simulink model "W07_pose_dp"  (R2024b)
settings: Solver=ode4  StartTime=0  StopTime=T_pose  FixedStep=h  RelTol=1e-3
InitFcn:
  | addpath(fullfile(fileparts(fileparts(fileparts(get_param(bdroot, 'FileName')))), '_tools'), fileparts(get_param(bdroot, 'FileName'))); run_alone('W07', bdroot);
StopFcn:
  | W07_plot_pose;
values from neighbouring files (symbols this model uses):
  alpha_lim = cfg.alpha_max(1)    [W07_0_setup.m]
  animate = 1    [W07_0_setup.m]    (also in W07_alloc_run.m = 0; W07_pose_run.m = 0; W07_wpt_run.m = 0)
  B_alloc = cfg.B    [W07_0_setup.m]
  beta_c = pi/2    (= 1.57079632679)    [W07_0_setup.m]
  eps_reg = 1e-4    (= 0.0001)    [W07_0_setup.m]    (also in W07_alloc_run.m)
  h = 0.02    [W07_0_setup.m]    (also in W07_3_build_wpt.m = add_line(sys, [a; via; b]); W07_4_build_pose.m = add_line(sys, [a; via; b]))
  k_neg = cfg.k_neg    [W07_0_setup.m]
  k_pos = cfg.k_pos    [W07_0_setup.m]
  Kb = 1    [W07_0_setup.m]
  Kd = 100    [W07_0_setup.m]
  Ki_u = 200    [W07_0_setup.m]
  Ki_v = 200    [W07_0_setup.m]
  Kp = 300    [W07_0_setup.m]
  Kp_pos = 0.30    (= 0.3)    [W07_0_setup.m]
  Kp_u = 200    [W07_0_setup.m]
  Kp_v = 200    [W07_0_setup.m]
  mp = 25    [W07_0_setup.m]
  N_lim = 150    [W07_0_setup.m]
  n_max = cfg.n_max    [W07_0_setup.m]    (also in W07_plot_ca.m = base_num('n_max',      103.93); W07_plot_sat.m = base_var('n_max',      103.931))
  n_min = cfg.n_min    [W07_0_setup.m]    (also in W07_plot_ca.m = base_num('n_min',     -101.74); W07_plot_sat.m = base_var('n_min',     -101.737))
  p_d = [10; 10]    [W07_0_setup.m]
  psi_set = deg2rad(45)    [W07_0_setup.m]
  Q_tau = eye(3)    [W07_0_setup.m]    (also in W07_alloc_run.m)
  quad = [cfg.pos ; cfg.alpha_max ; cfg.mount]    [W07_0_setup.m]
  rp = [0.05 0 -0.35]'    [W07_0_setup.m]
  T_neg = cfg.k_neg * cfg.n_min^2    [W07_0_setup.m]    (also in W07_plot_ca.m = base_num('T_neg',       66.708); W07_plot_sat.m = base_var('T_neg',        66.708))
  T_pos = cfg.k_pos * cfg.n_max^2    [W07_0_setup.m]    (also in W07_plot_ca.m = base_num('T_pos',      119.682); W07_plot_sat.m = base_var('T_pos',       119.682))
  u_lim = 0.80    (= 0.8)    [W07_0_setup.m]
  V_c = 0.0    (= 0)    [W07_0_setup.m]
  v_lim = 0.60    (= 0.6)    [W07_0_setup.m]
  W_alloc = diag(repmat([1 10], 1, 4))    [W07_0_setup.m]
  x0 = zeros(12,1)    [W07_0_setup.m]
  X_max = 120    [W07_0_setup.m]
  Y_max = 120    [W07_0_setup.m]
settings Model: Creator=admin  LastModifiedBy=admin
settings DataIOCC: ReturnWorkspaceOutputs=off

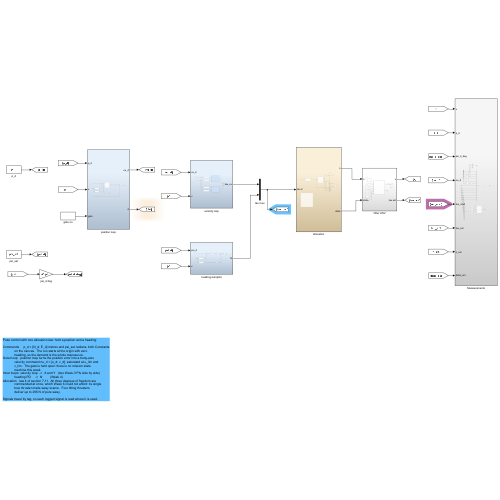
[thumbnail: Simulink's stored preview of the top-level diagram]
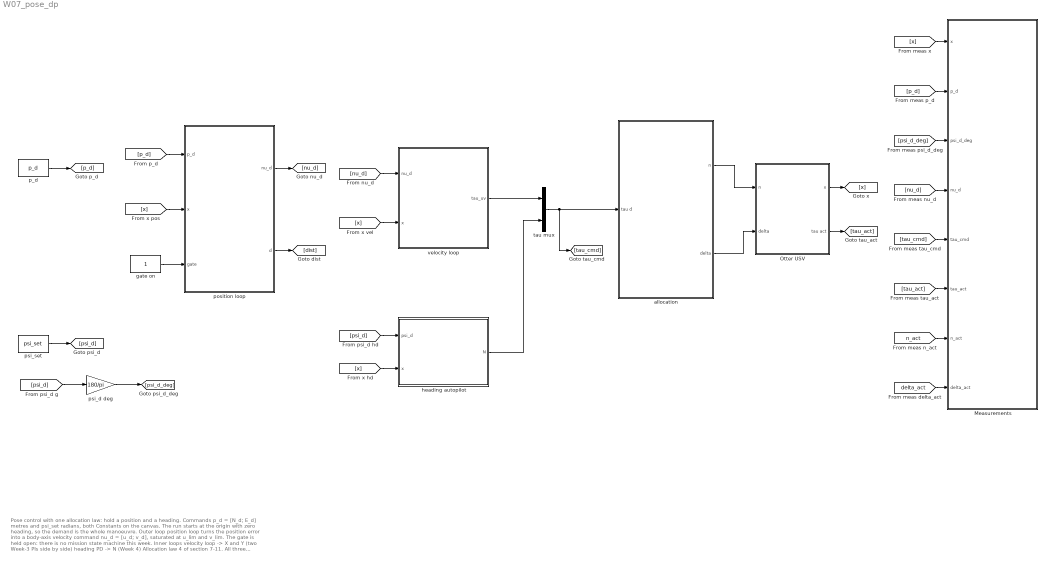
== system W07_pose_dp ==
  note: Pose control with one allocation law: hold a position and a heading.
      |
      | Commands     p_d = [N_d; E_d] metres and psi_set radians, both Constants
      |              on the canvas.  The run starts at the origin with zero
      |              heading, so the demand is the whole manoeuvre.
      | Outer loop   position loop turns the position error into a body-axis
      |              velocity command nu_d = [u_d; v_d], saturated at u_lim and
      |              v_lim.  The gate is held open: there is no mission state
      |              machine this week.
      | Inner loops  velocity loop  ->  X and Y   (two Week-3 PIs side by side)
      |              heading PD     ->  N         (Week 4)
      | Allocation   law 4 of section 7-11.  All three degrees of freedom are
      |              commanded at once, which Week 6 could not afford: its single
      |              bow thruster made sway scarce.  Four tilting thrusters
      |              deliver up to 295 N of pure sway.
      |
      | Signals travel by tag, so each logged signal is read where it is used.
  Measurements : Subsystem
  Otter USV : Subsystem
  allocation : Subsystem
  gate on : Constant
  heading autopilot : Subsystem
  p_d : Constant  Value=p_d
  position loop : Subsystem
  psi_d deg : Gain  Gain=180/pi
  psi_set : Constant  Value=psi_set
  tau mux : Mux  Inputs=2
  velocity loop : Subsystem
  wires:
  p_d/1 -> [p_d]
  psi_set/1 -> [psi_d]
  [psi_d] -> psi_d deg/1
  psi_d deg/1 -> [psi_d_deg]
  [p_d] -> position loop/1(p_d)
  [x] -> position loop/2(x)
  gate on/1 -> position loop/3(gate)
  position loop/1(nu_d) -> [nu_d]
  position loop/2(d) -> [dist]
  [nu_d] -> velocity loop/1(nu_d)
  [x] -> velocity loop/2(x)
  [psi_d] -> heading autopilot/1(psi_d)
  [x] -> heading autopilot/2(x)
  velocity loop/1(tau_uv) -> tau mux/1
  heading autopilot/1(N) -> tau mux/2
  tau mux/1 -> [tau_cmd], allocation/1(tau d)
  allocation/1(n) -> Otter USV/1(n)
  allocation/2(delta) -> Otter USV/2(delta)
  Otter USV/1(x) -> [x]
  Otter USV/2(tau act) -> [tau_act]
  [x] -> Measurements/1(x)
  [p_d] -> Measurements/2(p_d)
  [psi_d_deg] -> Measurements/3(psi_d_deg)
  [nu_d] -> Measurements/4(nu_d)
  [tau_cmd] -> Measurements/5(tau_cmd)
  [tau_act] -> Measurements/6(tau_act)
  [n_act] -> Measurements/7(n_act)
  [delta_act] -> Measurements/8(delta_act)

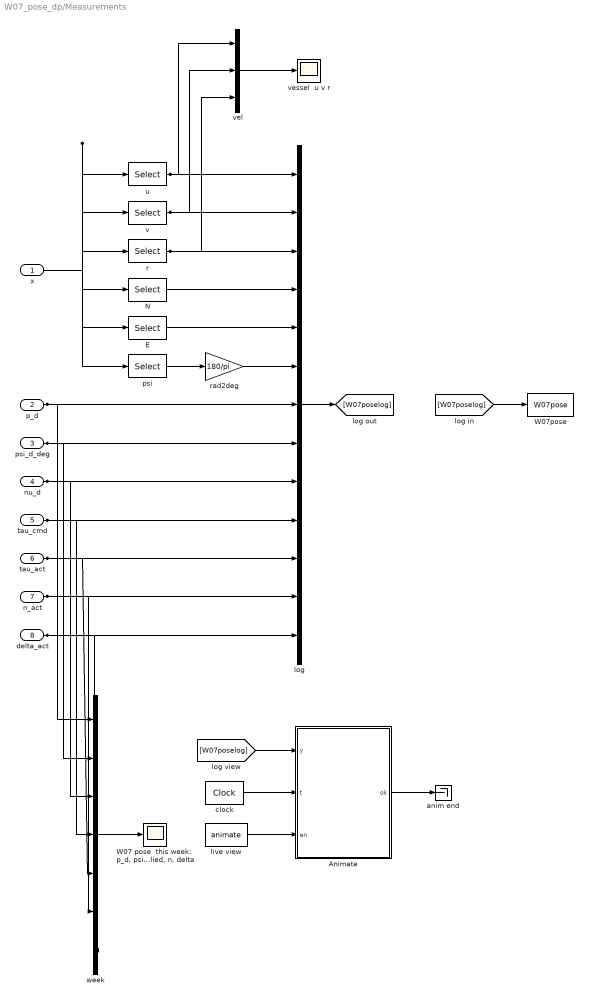
== system W07_pose_dp/Measurements ==
  x : Inport
  p_d : Inport  Port=2
  psi_d_deg : Inport  Port=3
  nu_d : Inport  Port=4
  tau_cmd : Inport  Port=5
  tau_act : Inport  Port=6
  n_act : Inport  Port=7
  delta_act : Inport  Port=8
  Animate : MATLAB Function  TreatAsAtomicUnit=on
  E : Selector  InputPortWidth=12  IndexOptions=Index vector (dialog)  Indices=8  OutputSizes=1
  N : Selector  InputPortWidth=12  IndexOptions=Index vector (dialog)  Indices=7  OutputSizes=1
  "W07 pose  this week:  p_d, psi_d, nu_d, tau asked and applied, n, delta" : Scope
  W07pose : ToWorkspace  VariableName=W07pose  SaveFormat=Structure With Time  SampleTime=-1
  anim end : Terminator
  clock : DigitalClock  SampleTime=h
  live view : Constant  Value=animate
  log : Mux  Inputs=13
  psi : Selector  InputPortWidth=12  IndexOptions=Index vector (dialog)  Indices=12  OutputSizes=1
  r : Selector  InputPortWidth=12  IndexOptions=Index vector (dialog)  Indices=6  OutputSizes=1
  rad2deg : Gain  Gain=180/pi
  u : Selector  InputPortWidth=12  IndexOptions=Index vector (dialog)  Indices=1  OutputSizes=1
  v : Selector  InputPortWidth=12  IndexOptions=Index vector (dialog)  Indices=2  OutputSizes=1
  vel : Mux  Inputs=3
  vessel  u v r : Scope
  week : Mux  Inputs=7
  wires:
  x/1 -> u/1, v/1, r/1, N/1, E/1, psi/1
  log/1 -> [W07poselog]
  [W07poselog] -> W07pose/1
  psi/1 -> rad2deg/1
  u/1 -> log/1, vel/1
  v/1 -> log/2, vel/2
  r/1 -> log/3, vel/3
  N/1 -> log/4
  E/1 -> log/5
  rad2deg/1 -> log/6
  p_d/1 -> log/7, week/1
  psi_d_deg/1 -> log/8, week/2
  nu_d/1 -> log/9, week/3
  tau_cmd/1 -> log/10, week/4
  tau_act/1 -> log/11, week/5
  n_act/1 -> log/12, week/6
  delta_act/1 -> log/13, week/7
  vel/1 -> vessel  u v r/1
  week/1 -> "W07 pose  this week:  p_d, psi_d, nu_d, tau asked and applied, n, delta"/1
  [W07poselog] -> Animate/1(y)
  clock/1 -> Animate/2(t)
  live view/1 -> Animate/3(en)
  Animate/1(ok) -> anim end/1

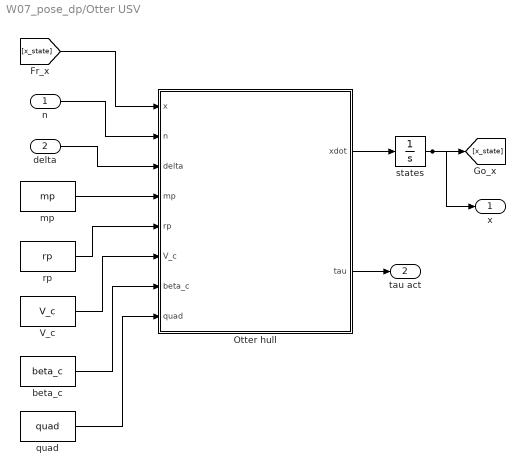
== system W07_pose_dp/Otter USV ==
  n : Inport
  delta : Inport  Port=2
  Otter hull : MATLAB Function  TreatAsAtomicUnit=on
  V_c : Constant  Value=V_c
  beta_c : Constant  Value=beta_c
  mp : Constant  Value=mp
  quad : Constant  Value=quad
  rp : Constant  Value=rp
  states : Integrator  InitialCondition=x0
  x : Outport
  tau act : Outport  Port=2
  wires:
  n/1 -> Otter hull/2(n)
  [x_state] -> Otter hull/1(x)
  delta/1 -> Otter hull/3(delta)
  mp/1 -> Otter hull/4(mp)
  rp/1 -> Otter hull/5(rp)
  V_c/1 -> Otter hull/6(V_c)
  beta_c/1 -> Otter hull/7(beta_c)
  quad/1 -> Otter hull/8(quad)
  Otter hull/1(xdot) -> states/1
  Otter hull/2(tau) -> tau act/1
  states/1 -> [x_state], x/1

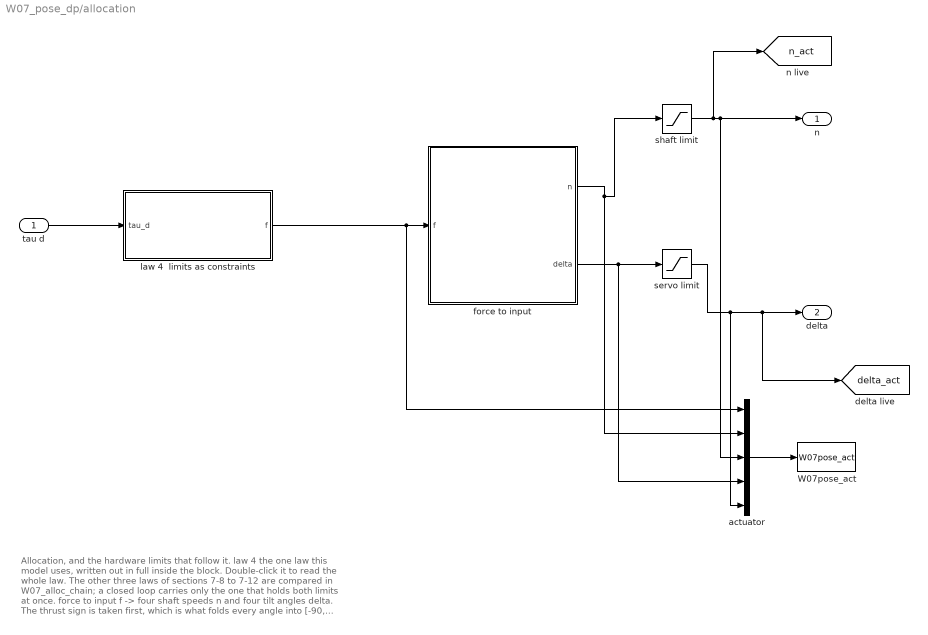
== system W07_pose_dp/allocation ==
  note: Allocation, and the hardware limits that follow it.
      |
      | law 4             the one law this model uses, written out in full
      |                   inside the block. Double-click it to read the whole law.
      |                   The other three laws of sections 7-8 to 7-12 are compared
      |                   in W07_alloc_chain; a closed loop carries only the one
      |                   that holds both limits at once.
      | force to input    f -> four shaft speeds n and four tilt angles delta. The
      |                   thrust sign is taken first, which is what folds every
      |                   angle into [-90, +90] deg before the servo ever sees it.
      |                   A unit asked for less than 0.5 N is held at n = 0 and
      |                   delta = 0, because below that the angle is arithmetic
      |                   noise and the servo would chatter at rest.
      | shaft limit       n clipped to [n_min, n_max].
      | servo limit       delta clipped to +-alpha_lim.
      | n live            the two clipped commands also leave as the global tags
      | delta live        n_act and delta_act, so the live view can draw them
      |                   against their limits while the run is still going. The
      |                   record below is readable only after it ends.
      | actuator          the record of this solve, written to W07pose_act as 24
      |                   columns:  f(8),  n asked(4),  n allowed(4),  delta
      |                   asked(4),  delta allowed(4). Wherever asked and allowed
      |                   differ, that unit is against a limit.
      |
      | What the hull was actually given is not rebuilt here: the motion model
      | already forms it from the clipped n and delta and reports it on its own
      | second output.
  tau d : Inport
  W07pose_act : ToWorkspace  VariableName=W07pose_act  SampleTime=-1
  actuator : Mux  Inputs=5
  force to input : MATLAB Function  TreatAsAtomicUnit=on
  law 4  limits as constraints : MATLAB Function  TreatAsAtomicUnit=on
  servo limit : Saturate  UpperLimit=alpha_lim  LowerLimit=-alpha_lim
  shaft limit : Saturate  UpperLimit=n_max  LowerLimit=n_min
  n : Outport
  delta : Outport  Port=2
  tag scope: delta_act=global, n_act=global
  wires:
  tau d/1 -> law 4  limits as constraints/1(tau_d)
  law 4  limits as constraints/1(f) -> force to input/1(f), actuator/1
  force to input/1(n) -> shaft limit/1, actuator/2
  force to input/2(delta) -> actuator/4, servo limit/1
  shaft limit/1 -> n/1, actuator/3, [n_act]
  servo limit/1 -> [delta_act], delta/1, actuator/5
  actuator/1 -> W07pose_act/1

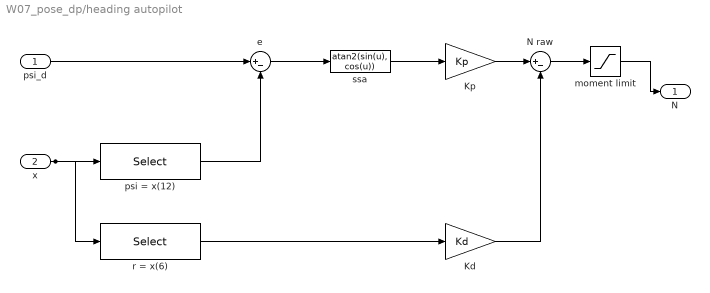
== system W07_pose_dp/heading autopilot ==
  psi_d : Inport
  x : Inport  Port=2
  Kd : Gain  Gain=Kd
  Kp : Gain  Gain=Kp
  N raw : Sum  Inputs=|+-
  e : Sum  Inputs=|+-
  moment limit : Saturate  UpperLimit=N_lim  LowerLimit=-N_lim
  psi = x(12) : Selector  InputPortWidth=12  IndexOptions=Index vector (dialog)  Indices=12  OutputSizes=1
  r = x(6) : Selector  InputPortWidth=12  IndexOptions=Index vector (dialog)  Indices=6  OutputSizes=1
  ssa : Fcn  Expr=atan2(sin(u), cos(u))
  N : Outport
  wires:
  x/1 -> psi = x(12)/1, r = x(6)/1
  psi_d/1 -> e/1
  psi = x(12)/1 -> e/2
  e/1 -> ssa/1
  ssa/1 -> Kp/1
  r = x(6)/1 -> Kd/1
  Kp/1 -> N raw/1
  Kd/1 -> N raw/2
  N raw/1 -> moment limit/1
  moment limit/1 -> N/1

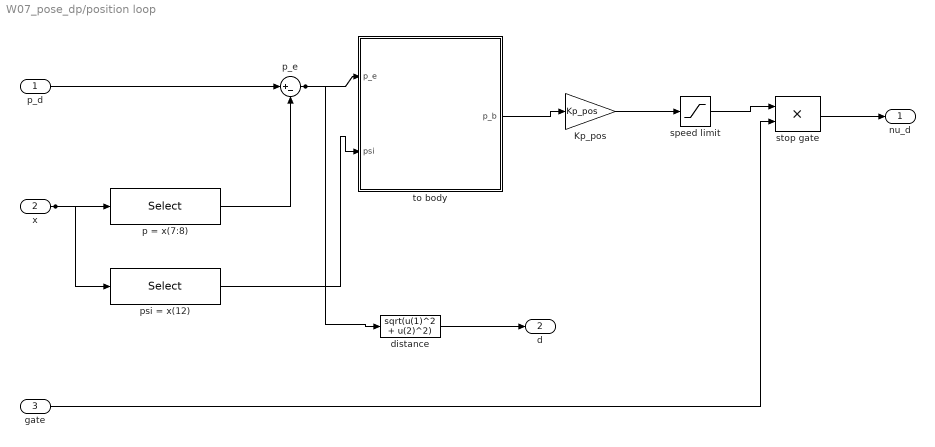
== system W07_pose_dp/position loop ==
  p_d : Inport
  x : Inport  Port=2
  gate : Inport  Port=3
  Kp_pos : Gain  Gain=Kp_pos
  distance : Fcn  Expr=sqrt(u(1)^2 + u(2)^2)
  p = x(7:8) : Selector  InputPortWidth=12  IndexOptions=Index vector (dialog)  Indices=[7 8]  OutputSizes=1
  p_e : Sum  Inputs=|+-
  psi = x(12) : Selector  InputPortWidth=12  IndexOptions=Index vector (dialog)  Indices=12  OutputSizes=1
  speed limit : Saturate  UpperLimit="[ u_lim;  v_lim]"  LowerLimit=[-u_lim; -v_lim]
  stop gate : Product
  to body : MATLAB Function  TreatAsAtomicUnit=on
  nu_d : Outport
  d : Outport  Port=2
  wires:
  x/1 -> p = x(7:8)/1, psi = x(12)/1
  p_d/1 -> p_e/1
  p = x(7:8)/1 -> p_e/2
  p_e/1 -> to body/1(p_e), distance/1
  psi = x(12)/1 -> to body/2(psi)
  to body/1(p_b) -> Kp_pos/1
  Kp_pos/1 -> speed limit/1
  speed limit/1 -> stop gate/1
  gate/1 -> stop gate/2
  stop gate/1 -> nu_d/1
  distance/1 -> d/1

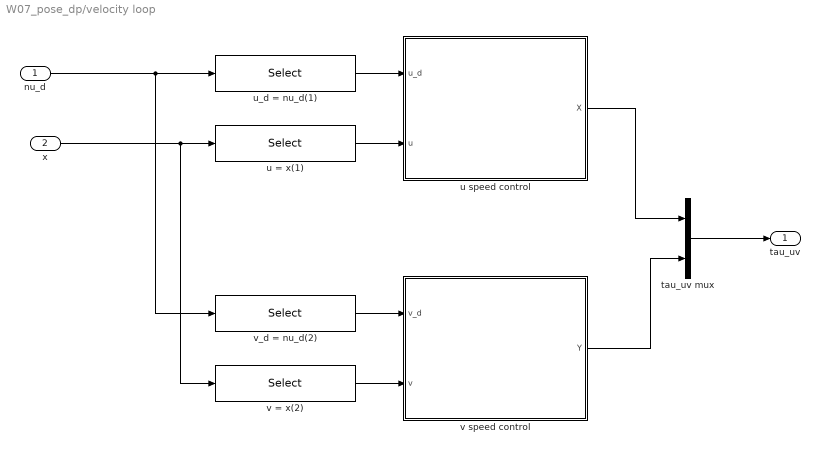
== system W07_pose_dp/velocity loop ==
  nu_d : Inport
  x : Inport  Port=2
  tau_uv mux : Mux  Inputs=2
  u = x(1) : Selector  InputPortWidth=12  IndexOptions=Index vector (dialog)  Indices=1  OutputSizes=1
  u speed control : Subsystem
  u_d = nu_d(1) : Selector  InputPortWidth=2  IndexOptions=Index vector (dialog)  Indices=1  OutputSizes=1
  v = x(2) : Selector  InputPortWidth=12  IndexOptions=Index vector (dialog)  Indices=2  OutputSizes=1
  v speed control : Subsystem
  v_d = nu_d(2) : Selector  InputPortWidth=2  IndexOptions=Index vector (dialog)  Indices=2  OutputSizes=1
  tau_uv : Outport
  wires:
  u_d = nu_d(1)/1 -> u speed control/1(u_d)
  u = x(1)/1 -> u speed control/2(u)
  v_d = nu_d(2)/1 -> v speed control/1(v_d)
  v = x(2)/1 -> v speed control/2(v)
  nu_d/1 -> u_d = nu_d(1)/1, v_d = nu_d(2)/1
  x/1 -> u = x(1)/1, v = x(2)/1
  u speed control/1(X) -> tau_uv mux/1
  v speed control/1(Y) -> tau_uv mux/2
  tau_uv mux/1 -> tau_uv/1

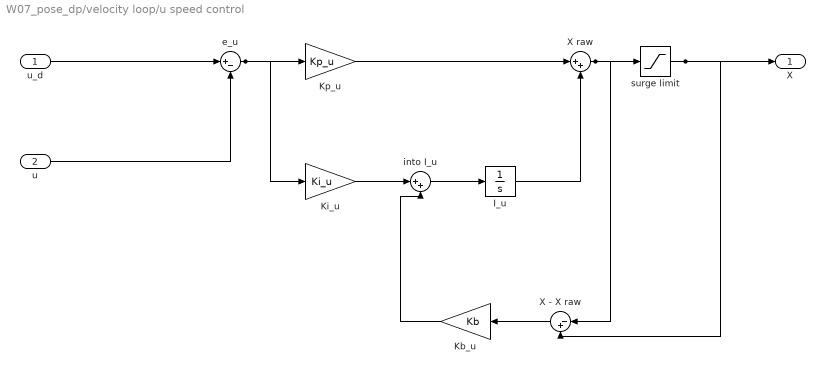
== system W07_pose_dp/velocity loop/u speed control ==
  u_d : Inport
  u : Inport  Port=2
  I_u : Integrator
  Kb_u : Gain  Gain=Kb
  Ki_u : Gain  Gain=Ki_u
  Kp_u : Gain  Gain=Kp_u
  X - X raw : Sum  Inputs=|-+
  X raw : Sum  Inputs=|++
  e_u : Sum  Inputs=|+-
  into I_u : Sum  Inputs=|++
  surge limit : Saturate  UpperLimit=X_max  LowerLimit=-X_max
  X : Outport
  wires:
  u_d/1 -> e_u/1
  u/1 -> e_u/2
  e_u/1 -> Kp_u/1, Ki_u/1
  Ki_u/1 -> into I_u/1
  into I_u/1 -> I_u/1
  Kp_u/1 -> X raw/1
  I_u/1 -> X raw/2
  X raw/1 -> surge limit/1, X - X raw/1
  surge limit/1 -> X - X raw/2, X/1
  X - X raw/1 -> Kb_u/1
  Kb_u/1 -> into I_u/2

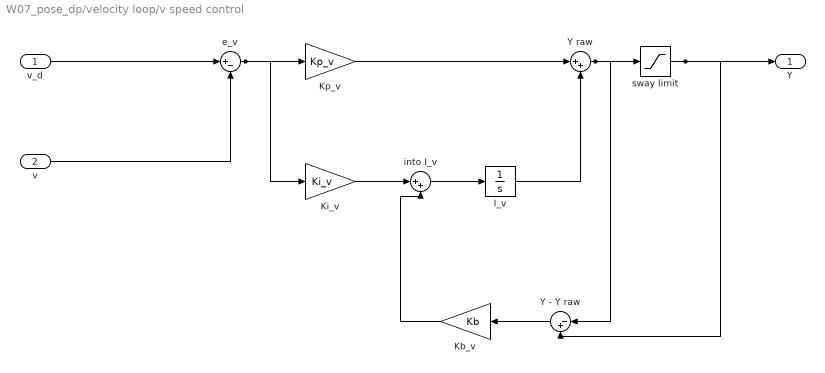
== system W07_pose_dp/velocity loop/v speed control ==
  v_d : Inport
  v : Inport  Port=2
  I_v : Integrator
  Kb_v : Gain  Gain=Kb
  Ki_v : Gain  Gain=Ki_v
  Kp_v : Gain  Gain=Kp_v
  Y - Y raw : Sum  Inputs=|-+
  Y raw : Sum  Inputs=|++
  e_v : Sum  Inputs=|+-
  into I_v : Sum  Inputs=|++
  sway limit : Saturate  UpperLimit=Y_max  LowerLimit=-Y_max
  Y : Outport
  wires:
  v_d/1 -> e_v/1
  v/1 -> e_v/2
  e_v/1 -> Kp_v/1, Ki_v/1
  Ki_v/1 -> into I_v/1
  into I_v/1 -> I_v/1
  Kp_v/1 -> Y raw/1
  I_v/1 -> Y raw/2
  Y raw/1 -> sway limit/1, Y - Y raw/1
  sway limit/1 -> Y - Y raw/2, Y/1
  Y - Y raw/1 -> Kb_v/1
  Kb_v/1 -> into I_v/2

== matlab function W07_pose_dp/allocation/law 4  limits as constraints ==
  data: tau_d input; f output double size=[8 1]; B_alloc parameter; W_alloc parameter; alpha_lim parameter; Q_tau parameter; eps_reg parameter; T_pos parameter; T_neg parameter
function f = law4_limits_as_constraints(tau_d, B_alloc, W_alloc, alpha_lim, Q_tau, eps_reg, T_pos, T_neg)
% LAW 4 -- the servo limit AND the thrust cap as hard constraints.  7-12.
%
% Minimise   ||Q (B f - tau_d)||^2 + eps ||W^(1/2) f||^2
% subject to, for every unit i,
%
%     |f_yi| <= tan(alpha_lim) sigma_i f_xi               the servo limit
%     cos(th) x' + sin(th) y' <= R cos(alpha_lim/M)       the thrust cap
%
% written in unit axes x' = sigma_i f_xi and y' = sigma_i f_yi. Both are
% straight lines once the thrust sign sigma_i of that unit is fixed, so the
% problem is a QP: no local minima. The signs are not known in advance, so
% all 2^4 = 16 sign combinations are solved and the cheapest feasible one is
% kept. tau_d sits in the cost rather than in an equality, so a solution
% exists even when the demand cannot be delivered.
%
% The cap is an arc, which no QP can hold. It is replaced by M = 3 inscribed
% chords: neighbouring chords meet exactly on the circle of radius R and
% their midpoints sit at cos(15 deg) = 0.966 R, so the polygon never breaks
% the cap and is at worst 3.4 per cent conservative.
%
% lsqlin has no code generation support, so the call is extrinsic and every
% output it returns is given a size and a type beforehand.
coder.extrinsic('lsqlin', 'optimoptions');

M = 3;                   % chords per cone, the n_chord of W07_vars
t = tan(alpha_lim);

% the whole cost as one least-squares residual,  ||C f - d||
C = [Q_tau*B_alloc ; sqrt(eps_reg)*sqrt(W_alloc)];
d = [Q_tau*tau_d   ; zeros(8,1)];

% the fallback, used if no sign combination turns out to be feasible
Wi = W_alloc \ eye(8);
f  = Wi * B_alloc' * ((B_alloc*Wi*B_alloc') \ tau_d);

opts = optimoptions('lsqlin', 'Display', 'off');
best = inf;

for p = 0:15
    % the four thrust signs of combination p, read off its four bits
    sg = zeros(4,1);
    for i = 1:4
        sg(i) = 1 - 2*mod(floor(p/2^(i-1)), 2);
    end

    A = zeros(4*(2+M), 8);
    b = zeros(4*(2+M), 1);
    r = 0;
    for i = 1:4
        s = sg(i);
        if s > 0
            R = T_pos;
        else
            R = T_neg;    % written positive, so the cap is a radius
        end
        r = r + 1;  A(r, 2*i-1) = -t*s;  A(r, 2*i) =  1;
        r = r + 1;  A(r, 2*i-1) = -t*s;  A(r, 2*i) = -1;
        for j = 1:M
            th = -alpha_lim + (j - 0.5)*(2*alpha_lim/M);
            r  = r + 1;
            A(r, 2*i-1) = s*cos(th);
            A(r, 2*i)   = s*sin(th);
            b(r)        = R*cos(alpha_lim/M);
        end
    end

    x   = zeros(8,1);
    cst = 0;
    res = zeros(11,1);
    ef  = 0;
    [x, cst, res, ef] = lsqlin(C, d, A, b, [], [], [], [], [], opts);

    % a cost is a cost only where the solver reported a solution
    if ef > 0 && cst < best
        best = cst;
        f    = x;
    end
end
end

== matlab function W07_pose_dp/position loop/to body ==
  data: p_e input; p_b output double size=[2 1]; psi input
function p_b = to_body(p_e, psi)
% Rotate the position error from NED into the body frame.
%
%            [ cos(psi)  -sin(psi) ]
%   R(psi) = [ sin(psi)   cos(psi) ]     maps the BODY frame to NED,
%
% so the transpose maps NED to the body frame. R is orthogonal, so the
% transpose is the inverse and nothing is lost in the change of frame: the
% distance to the target is the same number in either one.
c = cos(psi);
s = sin(psi);
p_b = [  c*p_e(1) + s*p_e(2) ;      % 전진 방향의 오차 / along the bow
        -s*p_e(1) + c*p_e(2) ];     % 우현 방향의 오차 / to starboard
end

== matlab function W07_pose_dp/allocation/force to input ==
  data: f input; n output double size=[4 1]; delta output; k_pos parameter; k_neg parameter
function [n, delta] = force2input(f, k_pos, k_neg)
% Eight force components -> four shaft speeds and four tilt angles.
%
%     sigma_i = sign(f_xi)                        which way the unit pushes
%     T_i     = sigma_i |f_i|                     signed thrust        [N]
%     delta_i = atan2(sigma_i f_yi, sigma_i f_xi) tilt angle         [rad]
%     n_i     = sign(T_i) sqrt(|T_i| / k_i)       shaft speed      [rad/s]
%
% Multiplying BOTH arguments of atan2 by sigma_i turns the direction through
% exactly pi, and because sigma_i f_xi >= 0 the result always lands in
% [-pi/2, +pi/2]. That is what keeps the angle reachable: a unit pushing
% astern comes out as negative thrust at a small angle instead of positive
% thrust at 180 deg, which no servo limited to +-45 deg could hold.
fx = f(1:2:7);
fy = f(2:2:8);
s  = sign(fx);
s(s == 0) = 1;      % a unit with no surge component is left pointing abeam

T     = s .* hypot(fx, fy);
delta = atan2(s.*fy, s.*fx);

% The coefficient depends on the sign because a propeller pushing astern is
% less efficient than the same propeller pushing ahead.
k = k_pos*double(T >= 0) + k_neg*double(T < 0);
n = sign(T) .* sqrt(abs(T) ./ k);

% Below a tiny force the angle stops meaning anything: atan2 of two numbers
% near zero turns with the last bit of the arithmetic, so a servo asked to
% follow it would chatter while the vessel sits still. Hold such a unit at
% zero instead. The threshold is 0.5 N, which is 0.4 % of the ahead cap, so
% no force a controller could usefully ask for is thrown away here.
tiny = hypot(fx, fy) < 0.5;
delta(tiny) = 0;
n(tiny)     = 0;
end

== matlab function W07_pose_dp/Otter USV/Otter hull ==
  data: x input; xdot output double size=[12 1]; n input; delta input; mp input; rp input; V_c input; beta_c input; quad input; tau output double size=[3 1]
function [xdot, tau] = otter_hull(x, n, delta, mp, rp, V_c, beta_c, quad)
% otter_tilt4.m: Fossen's otter.m with four tilting thrusters, called
% unchanged from _tools. Four shaft speeds and four angles in, tau built
% inside, in the same four marked places as otter_bow.m.
%
%   x      12 states, fed back from the integrator
%   n      shaft speeds [rad/s], fore port / fore stbd / aft port / aft stbd
%   delta  tilt angles [rad], measured from the body x axis, CCW positive
%   quad   3 x 4: the x stations, the y stations and the tilt limits
%
% Rows 1, 2 and 6 of tau all carry the angles, by the column rule
% [e_x; e_y; x e_y - y e_x] with e = [cos delta; sin delta]. Nothing is
% added after the call; there is no superposition and no tau_ext port.
%
% The second output is the [X; Y; N] the model actually used, formed after n
% and delta are clipped to their limits. It is the delivered force, so no
% block outside has to rebuild it from n and delta.
%
% otter_tilt4.m is not written for code generation, so the call is extrinsic
% and both outputs have to be pre-sized for Simulink to know their widths.
coder.extrinsic('otter_tilt4');

xdot = zeros(12,1);
spd  = 0;
tau  = zeros(3,1);
[xdot, spd, tau] = otter_tilt4(x, n, delta, mp, rp, V_c, beta_c, quad);
end

== matlab function W07_pose_dp/Measurements/Animate ==
  data: y input; ok output; t input; en input
function ok = Animate(y, t, en)
%#codegen
% Live view of the vessel while the model runs.
%
% A MATLAB Function block cannot plot, so the drawing function is declared
% extrinsic: Simulink calls plain MATLAB rather than generating code for it.
% Set animate = 0 in the setup script to switch the live view off.
%
% y is the whole log vector, in the column order this subsystem builds:
% [u v r N E psi] first, psi in DEGREES, then the week's own signals.
% The wrapper names the columns; nothing else counts them.
coder.extrinsic('W07pose_animate');
ok = 1;
if en > 0.5
    W07pose_animate(y, t);
end
end
